simulink model "PSO_BON"  (R2019b)
settings: Solver=VariableStepAuto  StartTime=0.0  StopTime=0.2  RelTol=1e-5
undefined symbols (not defined in the file): sigbuilder_block
libraries: powerlib x164, re_lib x96, powerlib_meascontrol x9
(part 5 of 6)

== matlab function PSO_BON/Phasor PSO1/MATLAB Function1 ==
  settings: updateMethod=DISCRETE  sampleTime=1e-4
  data: Vpv input; Duty output; Ipv input
function Duty = PPSO(Vpv,Ipv)
coder.extrinsic('rand')
coder.extrinsic('format long')

persistent v_2 vmax_2 delta_2 iter_2 count_Part_2 count_2 pos_2 fitness_2 fitnessPbest_2 Pbest_2 fitnessGbest_2 Gbest_2 count_conv_2 reinit_2 Duty_Init_2;
Npart = 5;              % Nombre de particules de l'éssain
maxiter = 10000000;     % Nombre d'itération
% D = 1;                  % nombre d'espace de recherche

% Espace de recherche
% ------------------------------------
duty_cl_min = 0.1;      % Valeur minimale du rapport cyclique
duty_cl_max = 0.9;      % Valeur maximale du rapport cyclique

% Tolérance de la puissance
% ------------------------------------
tolerance = 1;          % Tolerance de la puissance en sortie

% Initialisation des vitesses des particules
% -------------------------------------------
if(isempty(vmax_2))
    vmax_2 = 0.5*(duty_cl_max - duty_cl_min);
end

if(isempty(v_2))
    v_2 = zeros(Npart,1);
end

% Initialisation de delta
% -------------------------------------------
if(isempty(delta_2))
    delta_2 = unifrnd(0,2*pi);
end

% Initialisation des positions des particules
% -------------------------------------------  
r = zeros(Npart,1);
r = rand(Npart,1);
if(isempty(pos_2))                                                          % Si la position des particules est inexistant
    pos_2 = zeros(Npart,1);
    for i = 1:Npart-2
        Min = duty_cl_min + (i-1)*(duty_cl_max-duty_cl_min)/(Npart-2);
        Max = Min + (duty_cl_max-duty_cl_min)/(Npart-2);
        pos_2(i+1) = Min + r(i)*(Max-Min);
%         pos_2(i) = duty_cl_min + ((duty_cl_max-duty_cl_min)*(i-1))/(Npart-1);
    end
    pos_2(1) = duty_cl_min;
    pos_2(Npart) = duty_cl_max;
end

% Initialisation des parametres persitents
% -------------------------------------------------
if(isempty(iter_2))       % Si le numéro de l'iteration est inexistant fixe à 1
    iter_2 = 1;
end

if(isempty(fitness_2))    % Si la fonction cout des particules est inexistant
    fitness_2 = zeros(Npart,1);
end

if(isempty(fitnessPbest_2))   % Si les fonctions couts des meilleures positions des particules est inexistant
    fitnessPbest_2 = zeros(Npart,1);
end

if(isempty(Pbest_2))      % Si les meilleures positions des particules est inexistant
    Pbest_2 = zeros(Npart,1);
end

if(isempty(Gbest_2))      % Si la meilleure position de l'éssain est inexistant
    Gbest_2 = zeros(maxiter,1);
end

if(isempty(fitnessGbest_2))   % Si la fonction cout de la meilleure position de l'éssain est inexistant
    fitnessGbest_2 = zeros(maxiter,1);
end

if(isempty(count_Part_2)) % Si le compteur de particule est inexistant
    count_Part_2 = 1;
end

if(isempty(count_conv_2)) % Si le compteur de particule convergente est inexistant
    count_conv_2 = zeros(Npart,1);
end

if(isempty(reinit_2))   % Si le coefficeint de reinitialisation est inexistant
    reinit_2 = 0;
end

if(isempty(Duty_Init_2))
    Duty_Init_2 = 0;
end

if(isempty(count_2))      % Si le compteur du régime transitoire est inexistant
    count_2 = 1;
end


% Evaluation des particules initiales
% -------------------------------------------------

%% phase transitoire d'évaluation d'une particule
% -------------------------------------------------
if (count_2 >= 1 && count_2 <= 20)
    Duty = pos_2(count_Part_2);
    count_2 = count_2 + 1;

    %% En cas de convergence
    % ---------------------------------------------
    if (reinit_2 == 1)  
        fitnessGbest_2(iter_2) = Vpv*Ipv;
        Duty = Duty_Init_2;
            if (abs(fitnessGbest_2(iter_2) - fitnessGbest_2(iter_2-1)) < 1)
                count_2 = count_2 - 1;
                reinit_2 = 1;
            else
                reinit_2 = 0;
                r = zeros(Npart,1);
                r = rand(Npart,1);
                pos_2 = zeros(Npart,1);
                for i = 1:Npart-2
                    Min = duty_cl_min + (i-1)*(duty_cl_max-duty_cl_min)/(Npart-2);
                    Max = Min + (duty_cl_max-duty_cl_min)/(Npart-2);
                    pos_2(i+1) = Min + r(i)*(Max-Min);
                end
                pos_2(1) = duty_cl_min;
                pos_2(Npart) = duty_cl_max;
                iter_2 = 0;
                vmax_2 = 0.5*(duty_cl_max - duty_cl_min);
                v_2 = zeros(Npart,1);
                delta_2 = unifrnd(0,2*pi);
                fitness_2 = zeros(Npart,1);
                fitnessPbest_2 = zeros(Npart,1);
                Pbest_2 = zeros(Npart,1);
                Gbest_2 = zeros(maxiter,1);
                fitnessGbest_2 = zeros(maxiter,1);
                count_Part_2 = 1;
                count_conv_2 = zeros(Npart,1);
                Duty_Init_2 = 0;
                count_2 = 1;
                iter_2 = iter_2 + 1;
            end 
    end
    return;
    
%%
else
    if(count_Part_2 <= (Npart - 1))
        Duty = pos_2(count_Part_2 + 1);
    else
        Duty = pos_2(1);
    end
end
                        % Programme PSO principale ou se fait la
                        % mise à jour des Pbest, de Gbest, des vitesse et
                        % des positions des particules
                        % -------------------------------------------------
fitness_2(count_Part_2) = Vpv*Ipv;  % Fonction cout des particules
if (count_Part_2 <= (Npart - 1))
    count_Part_2 = count_Part_2 + 1;
    count_2 = 2;
else
    if (iter_2 == 1)
                        % Initialisation des Pbest
                        % -------------------------------------------------
%         for j = 1:D
            for i = 1:Npart
                Pbest_2(i) = pos_2(i);
                fitnessPbest_2(i) = fitness_2(i);
            end
%         end
                        % Détermination de la fonction cout maximale
                        % -------------------------------------------------
        maxFitnessPbest = 0;
        FitnessPbest = fitnessPbest_2(:);
        for j = 1:length(FitnessPbest)
            if FitnessPbest(j) > maxFitnessPbest
                maxFitnessPbest = FitnessPbest(j);
            end
        end
                        % Initialisation de Gbest
                        % -------------------------------------------------
        fitnessGbest_2(iter_2) = maxFitnessPbest;
%         for i = 1:D
            for k = 1:Npart
                if(fitnessGbest_2(iter_2) == fitnessPbest_2(k))
                    Gbest_2(iter_2) = Pbest_2(k);
                end
            end
%         end
    elseif (iter_2 >= 2 && iter_2 <= maxiter)
                        % Mise à jour des Pbest
                        % -------------------------------------------------
%         for j = 1:D
            for i = 1:Npart
                if (fitness_2(i) > fitnessPbest_2(i))
                    Pbest_2(i) = pos_2(i);
                    fitnessPbest_2(i) = fitness_2(i);
                end
            end
%         end
                        % Mise à jour de Gbest
                        % -------------------------------------------------
        maxFitnessPbest = 0;
        FitnessPbest = fitnessPbest_2(:);
        for j = 1:length(FitnessPbest)
            if FitnessPbest(j) > maxFitnessPbest
                maxFitnessPbest = fitnessPbest_2(j);
            end
        end
        fitnessGbest_2(iter_2) = maxFitnessPbest;
%         for i = 1:D
            for k=1:Npart
                if(fitnessGbest_2(iter_2) == fitnessPbest_2(k))
                    Gbest_2(iter_2) = Pbest_2(k);
                end
            end
%         end
    end
                       % Test de convergence
                        % -------------------------------------------------
%     for j = 1:D
        for i = 1:Npart
            if ((fitnessGbest_2(iter_2) - fitnessPbest_2(i)) < tolerance)
                count_conv_2(i) = 1;
            end
        end
%     end
    n = sum(count_conv_2);
    if (n == Npart)
        reinit_2 = 1;
        Duty_Init_2 = Gbest_2(iter_2);
    else
        count_conv_2 = zeros(Npart,1);
    end
                        % Mise à jour des positions et des vitesses des
                        % particules
                        % -------------------------------------------------
        aa=2*(sin(delta_2));
        bb=2*(cos(delta_2));
        ee=abs(cos(delta_2))^aa;
        tt=abs(sin(delta_2))^bb;
    for i = 1:Npart
        v_2(i) = (ee)*(Pbest_2(i) - pos_2(i)) + (tt)*(Gbest_2(iter_2) - pos_2(i));
        if (v_2(i) > vmax_2)
            v_2(i) = vmax_2;
        end
        if (v_2(i) < -vmax_2)
            v_2(i) = -vmax_2;
        end
%         v_2(i) = min(max(v_2(i),-vmax_2),vmax_2);
        pos_2(i) = pos_2(i) + v_2(i);
        if (pos_2(i) > duty_cl_max)
            pos_2(i) = duty_cl_max;
        end
        if (pos_2(i) < duty_cl_min)
            pos_2(i) = duty_cl_min;
        end
%         pos_2(i) = min(max(pos_2(i),duty_cl_min),duty_cl_max);
    end
        delta_2 = delta_2 + (abs(aa + bb)*(2*pi));
        vmax_2 = (abs(cos(delta_2))^2)*(duty_cl_max - duty_cl_min);
                        % Mise à jour des positions et des vitesses
                        % -------------------------------------------------

                        % Contraindre la position mise à jour dans
                        % l'intervale de recherche
                        % -------------------------------------------------
%     end
    pos_2
    Duty = pos_2(1);
    count_Part_2 = 1;
    count_2 = 2;
    iter_2 = iter_2 + 1;
    if iter_2 > maxiter
        iter_2 = maxiter;
    end
end
end

== matlab function PSO_BON/Variant PSO1/MATLAB Function1 ==
  settings: updateMethod=DISCRETE  sampleTime=1e-4
  data: Vpv input; D output; Ipv input
function D = PSO(Vpv,Ipv)
%#codegen
persistent u;
persistent dcurrent;
persistent pbest;
persistent p;
persistent dc;
persistent v;
persistent counter;
persistent gbest;
Npart = 10;
if(isempty(counter))
    counter=0;
end
if(isempty(dcurrent))
    dcurrent=0.5;
end
if(isempty(gbest))
    gbest=0.5;
end
if(isempty(p))
    p=zeros(Npart,1);
end

if(isempty(v))
    v=zeros(Npart,1);
end

if(isempty(pbest))
    pbest=zeros(Npart,1);
end
if(isempty(u))
    u=0;
end
if(isempty(dc))
    dc=zeros(Npart,1);
    dc(1)=0;
    dc(2)=0.1;
    dc(3)=0.2;
    dc(4)=0.3;
    dc(5)=0.4;
    dc(6)=0.5;
    dc(7)=0.6;
    dc(8)=0.7;
    dc(9)=0.8;
    dc(10)=0.9;
end
if(counter>=1 && counter<20)
    D=dcurrent;
    counter=counter+1;
    return;
end
counter=0;

if(u>=1 && u<=Npart)
    if((Vpv*Ipv)>p(u))
        p(u)=Vpv*Ipv;
        pbest(u)=dcurrent;
    end
end
u=u+1;
if(u==Npart+2)
    u=1;
end
if(u==1)
    D=dc(u);
    dcurrent=D;
    counter=1;
    return;
elseif(u==2)
    D=dc(u);
    dcurrent=D;
    counter=1;
    return;
elseif(u==3)
    D=dc(u);
    dcurrent=D;
    counter=1;
    return;
elseif(u==4)
    D=dc(u);
    dcurrent=D;
    counter=1;
    return;
elseif(u==5)
    D=dc(u);
    dcurrent=D;
    counter=1;
    return;
elseif(u==6)
    D=dc(u);
    dcurrent=D;
    counter=1;
    return;
elseif(u==7)
    D=dc(u);
    dcurrent=D;
    counter=1;
    return;
elseif(u==8)
    D=dc(u);
    dcurrent=D;
    counter=1;
    return;
elseif(u==9)
    D=dc(u);
    dcurrent=D;
    counter=1;
    return;
elseif(u==10)
    D=dc(u);
    dcurrent=D;
    counter=1;
    return;
elseif(u==Npart+1)
    [m,i]=max(p);
    gbest=pbest(i);
    D=gbest;
    dcurrent=D;
    counter=1;
    %update velocity and duty cycle
    v(1)=updatevelocity(v(1),pbest(1),dc(1),gbest)
    v(2)=updatevelocity(v(2),pbest(2),dc(2),gbest)
    v(3)=updatevelocity(v(3),pbest(3),dc(3),gbest)
    v(4)=updatevelocity(v(4),pbest(4),dc(4),gbest)
    v(5)=updatevelocity(v(5),pbest(5),dc(5),gbest)
    v(6)=updatevelocity(v(6),pbest(6),dc(6),gbest)
    v(7)=updatevelocity(v(7),pbest(7),dc(7),gbest)
    v(8)=updatevelocity(v(8),pbest(8),dc(8),gbest)
    v(9)=updatevelocity(v(9),pbest(9),dc(9),gbest)
    v(10)=updatevelocity(v(10),pbest(10),dc(10),gbest)
    %update duty cycle
    dc(1)=updateduty(dc(1),v(1))
    dc(2)=updateduty(dc(2),v(2))
    dc(3)=updateduty(dc(3),v(3))
    dc(4)=updateduty(dc(4),v(4))
    dc(5)=updateduty(dc(5),v(5))
    dc(6)=updateduty(dc(6),v(6))
    dc(7)=updateduty(dc(7),v(7))
    dc(8)=updateduty(dc(8),v(8))
    dc(9)=updateduty(dc(9),v(9))
    dc(10)=updateduty(dc(10),v(10))
    return;
    
else
    u
    y='hello'
    D=0.1
    
end


end
function vfinal=updatevelocity(velocity,pobest,d,gwbest)
% PSO Parameters
w=0.4;
c1=1.2;       % Personal Learning Coefficient
c2=2;         % Global Learning Coefficient
beta = 1.5;
%w=(1.1-(pobest/gwbest));            % Inertia Weight
             % Inertia Weight Damping Ratio
% If you would like to use Constriction Coefficients for PSO,
% uncomment the following block and comment the above set of parameters.

% % Constriction Coefficients
% phi1=2.05;
% phi2=2.05;
% phi=phi1+phi2;
% chi=2/(phi-2+sqrt(phi^2-4*phi));
% w=chi;          % Inertia Weight
% wdamp=1;        % Inertia Weight Damping Ratio
% c1=chi*phi1;    % Personal Learning Coefficient
% c2=chi*phi2;    % Global Learning Coefficient
% vfinal = (w*velocity)+(c1*rand(1)*(pobest-d))+(c2*rand(1)*(gwbest-d));
vfinal = (w*velocity)+beta*(gwbest-d);
end
function dfinal=updateduty(d,velocity)
dup=d+velocity;
if(dup>0.9)
    dfinal=0.9;
elseif(dup<0.1)
    dfinal=0.1;
else
    dfinal=dup;
end
end

== matlab function PSO_BON/Phasor PSO1/MATLAB Function2 ==
  settings: updateMethod=DISCRETE  sampleTime=1e-4
  data: Vpv input; D output; Ipv input; G output; P output; Pow output; Powb output; Pp output
function [D, G, P, Pow, Powb, Pp] = PSO_Mod(Vpv,Ipv)
coder.extrinsic('rand')
coder.extrinsic('format long')

persistent iter count_Part count pos fitness fitnessPbest Pbest fitnessGbest Gbest count_conv reinit Duty_Init;
Npart = 5;              % Nombre de particules de l'éssain
maxiter = 10000000;           % Nombre d'itération

% Espace de recherche
% ------------------------------------
duty_cl_min = 0.1;      % Valeur minimale du rapport cyclique
duty_cl_max = 0.9;      % Valeur maximale du rapport cyclique

% Tolérance de la puissance
% ------------------------------------
tolerance = 1;          % Tolerance de la puissance en sortie

% Initialisation des positions des particules
% ------------------------------------
r = zeros(Npart,1);     % génération d'un vecteur de nombre aléatoire compris entre 0 et 1
r = rand(Npart,1);      
if(isempty(pos))        % Si la position des particules est inexistant
    pos = zeros(Npart,1);
%     for i = 1:Npart
%         pos(i) = duty_cl_min + ((duty_cl_max-duty_cl_min)*(i-1))/(Npart-1);
% %         pos(i) = duty_cl_min + r(i)*(duty_cl_max-duty_cl_min);
%     end
    
    for i = 1:Npart-2
        Min = duty_cl_min + (i-1)*(duty_cl_max-duty_cl_min)/(Npart-2);
        Max = Min + (duty_cl_max-duty_cl_min)/(Npart-2);
        pos(i+1) = Min + r(i)*(Max-Min);
    end
    pos(1) = duty_cl_min;
    pos(Npart) = duty_cl_max;
    Pp = pos;
end

% Initialisation des parametres persitents
% -------------------------------------------------
if(isempty(iter))       % Si le numéro de l'iteration est inexistant fixe à 1
    iter = 1;
end
if(isempty(fitness))    % Si la fonction cout des particules est inexistant
    fitness = zeros(Npart,1);
end
if(isempty(fitnessPbest))   % Si les fonctions couts des meilleures positions des particules est inexistant
    fitnessPbest = zeros(Npart,1);
    Powb = fitnessPbest;
end
if(isempty(Pbest))      % Si les meilleures positions des particules est inexistant
    Pbest = zeros(Npart,1);
    P = Pbest;
end
if(isempty(Gbest))      % Si la meilleure position de l'éssain est inexistant
    Gbest = zeros(maxiter,1);
end
if(isempty(fitnessGbest))   % Si la fonction cout de la meilleure position de l'éssain est inexistant
    fitnessGbest = zeros(maxiter,1);
    Pow = fitnessGbest(iter);
end
if(isempty(count_Part)) % Si le compteur de particule est inexistant
    count_Part = 1;
end
if(isempty(count_conv)) % Si le compteur de particule convergente est inexistant
    count_conv = zeros(Npart,1);
end
if(isempty(reinit))   % Si le coefficeint de reinitialisation est inexistant
    reinit = 0;
end
if(isempty(Duty_Init))
    Duty_Init = 0;
end
if(isempty(count))      % Si le compteur du régime transitoire est inexistant
    count = 1;
end

% Evaluation des particules initiales
% -------------------------------------------------

%% phase transitoire d'évaluation d'une particule
% -------------------------------------------------
if (count >= 1 && count <= 20)
    D = pos(count_Part);
    G = Duty_Init;
    P = Pbest;
    Pow = fitnessGbest(iter);
    Powb = fitnessPbest;
    Pp = pos;
    count = count + 1;

    %% En cas de convergence
    % ---------------------------------------------
    if (reinit == 1)  
        fitnessGbest(iter) = Vpv*Ipv;
        D = Duty_Init;
        G = Duty_Init;
        P = Pbest;
        Pp = pos;
        iter;
        Pow = fitnessGbest(iter);
        Powb = fitnessPbest;
%         if iter < 15
            if (abs(fitnessGbest(iter) - fitnessGbest(iter-1)) < 1)
                count = count - 1;
                iter;
                reinit = 1;
                Pow = fitnessGbest(iter);
                Powb = fitnessPbest;
                Pp = pos;
                P = Pbest;
            else
                reinit = 0;
                pos = zeros(Npart,1);    
                for i = 1:Npart-2
                    Min = duty_cl_min + (i-1)*(duty_cl_max-duty_cl_min)/(Npart-2);
                    Max = Min + (duty_cl_max-duty_cl_min)/(Npart-2);
                pos(i+1) = Min + r(i)*(Max-Min);
                end
                pos(1) = duty_cl_min;
                pos(Npart) = duty_cl_max;
                Pp = pos;
                P = Pbest;
                iter = 1;
                fitness = zeros(Npart,1);
                fitnessPbest = zeros(Npart,1);
                Pbest = zeros(Npart,1);
                Gbest = zeros(maxiter,1);
                fitnessGbest = zeros(maxiter,1);
                count_Part = 1;
                count_conv = zeros(Npart,1);
                Duty_Init = 0;
                count = 1;
            end
%         else
%             if (abs(fitnessGbest(iter) - fitnessGbest(iter-10)) < 0.5)
%                 count = count - 1;
%                 reinit = 1;
%             else
%                 reinit = 0;
%                 pos = zeros(Npart,1);    
%                 for i = 1:Npart-2
%                     Min = duty_cl_min + (i-1)*(duty_cl_max-duty_cl_min)/(Npart-2);
%                     Max = Min + (duty_cl_max-duty_cl_min)/(Npart-2);
%                 pos(i+1) = Min + r(i)*(Max-Min);
%                 end
%                 pos(1) = duty_cl_min;
%                 pos(Npart) = duty_cl_max;
%                 Pp = pos;
%                 iter = 1;
%                 fitness = zeros(Npart,1);
%                 fitnessPbest = zeros(Npart,1);
%                 Pbest = zeros(Npart,1);
%                 Gbest = zeros(maxiter,1);
%                 fitnessGbest = zeros(maxiter,1);
%                 count_Part = 1;
%                 count_conv = zeros(Npart,1);
%                 Duty_Init = 0;
%                 count = 1;
%             end
%         end
%         iter = iter + 1;
%         G = 0;
%         GG = 1;
%         P = zeros(Npart,1);
%         Pp = pos;
%         count = count - 1;          % Décrémenter
        
    end
    return;
    
%%
else
    if(count_Part <= (Npart - 1))
        D = pos(count_Part + 1);
        G = Gbest(iter);
        P = Pbest;
        Pp = pos;
        Pow = fitnessGbest(iter);
        Powb = fitnessPbest;
    else
        D = pos(1);
        G = Gbest(iter);
        P = Pbest;
        Pp = pos;
        Pow = fitnessGbest(iter);
        Powb = fitnessPbest;
    end
end


Pp = pos;
                        % Programme PSO principale ou se fait la
                        % mise à jour des Pbest, de Gbest, des vitesse et
                        % des positions des particules
                        % -------------------------------------------------
fitness(count_Part) = Vpv*Ipv;  % Fonction cout des particules
if (count_Part <= (Npart - 1))
    count_Part = count_Part + 1;
    count = 2;
else
    pos;
    Pp = pos;
    if (iter == 1)
                        % Initialisation des Pbest
                        % -------------------------------------------------
        for i = 1:Npart
            Pbest(i) = pos(i);
            fitnessPbest(i) = fitness(i);
        end
        Pbest;
        fitnessPbest;
        P = Pbest;
        Pow = fitnessGbest(iter);
        Powb = fitnessPbest;
        Pp = pos;
                        % Détermination de la fonction cout maximale
                        % -------------------------------------------------
        maxFitnessPbest = 0;
        for j = 1:length(fitnessPbest)
            if fitnessPbest(j) > maxFitnessPbest
                maxFitnessPbest = fitnessPbest(j);
            end
        end
                        % Initialisation de Gbest
                        % -------------------------------------------------
        fitnessGbest(iter) = maxFitnessPbest;
        for k = 1:Npart
            if(fitnessGbest(iter) == fitnessPbest(k))
                Gbest(iter) = Pbest(k);
            end
        end
    elseif (iter >= 2 && iter <= maxiter)
                        % Mise à jour des Pbest
                        % -------------------------------------------------
        for i = 1:Npart
            if (fitness(i) > fitnessPbest(i))
                Pbest(i) = pos(i);
                fitnessPbest(i) = fitness(i);
            end
        end
        Pbest;
        fitnessPbest;
        P = Pbest;
        Pow = fitnessGbest(iter);
        Powb = fitnessPbest;
        Pp = pos;
                        % Mise à jour de Gbest
                        % -------------------------------------------------
        maxFitnessPbest = 0;
        for j = 1:length(fitnessPbest)
            if fitnessPbest(j) > maxFitnessPbest
                maxFitnessPbest = fitnessPbest(j);
            end
        end
        fitnessGbest(iter) = maxFitnessPbest;
        for k=1:Npart
            if(fitnessGbest(iter) == fitnessPbest(k))
                Gbest(iter) = Pbest(k);
%                 G = Gbest(iter);
            end
        end
    end
    G = Gbest(iter);
                       % Test de convergence
                        % -------------------------------------------------
    for i = 1:Npart
        if ((fitnessGbest(iter) - fitnessPbest(i)) < tolerance)
            count_conv(i) = 1;
        end
    end
    n = sum(count_conv);
    if (n == Npart)
        reinit = 1;
        Duty_Init = Gbest(iter);
        G = Gbest(iter);
    else
        count_conv = zeros(Npart,1);
        G = Gbest(iter);
    end
                        % Mise à jour des positions et des vitesses des
                        % particules
                        % -------------------------------------------------
    for i = 1:Npart
                        % Mise à jour des positions sur le principe de la
                        % dichotomie
                        % -------------------------------------------------
%         if Gbest(iter) == Pbest(i)
%             pos(i) = Pbest(i) + 0.001;
%         else
            pos(i) = (Gbest(iter)+pos(i))/2;
%         end
                        % Contraindre la position mise à jour dans
                        % l'intervale de recherche
                        % -------------------------------------------------
        if (pos(i) > duty_cl_max)
            pos(i) = duty_cl_max;
        end
        if (pos(i) < duty_cl_min)
            pos(i) = duty_cl_min;
        end
    end
    pos;
    D = pos(1);
    iter
    reinit
    G = Gbest(iter);
    P = Pbest
    Pow = fitnessGbest(iter)
    Powb = fitnessPbest
    Pp = pos;
    count_Part = 1;
    count = 2;
    iter = iter + 1;
    if iter > maxiter
        iter = maxiter;
    end
end
end

== matlab function PSO_BON/InCond1/MATLAB Function1 ==
  settings: updateMethod=DISCRETE  sampleTime=1e-4
  data: V input; D output; I input
% InCond
function D= InCond(V,I)
delta=0.005;
Dmax = 0.9;   %Maximum value for D
Dmin = 0.1;   %Minimum value for D

persistent V0 I0 D0;
if isempty(V0)
    V0=0; I0=0; D0=0.5;
end
%-------------------------------------
m=0;
dV=V-V0; dI=I-I0; 
if dV==0             % Si no hay cambio voltaje
	  if dI==0
		 m=D0;
	  else
		if dI>0
		  m=D0-delta;
		else
		  m=D0+delta;
		end
	  end
elseif	dI/dV==-(I/V)   %no hacer nada (MPP)
else                    %dI/dV~=-(I/V)
        if dI/dV>-(I/V) %dI/dV>-(I/V) (izquierda MPP)
           m=D0-delta;  %disminuir D
        else            %dI/dV<-(I/V) (derecha MPP)
           m=D0+delta;  %aumentar D
        end 
end
D=m;
%-------------------------------------
if D >= Dmax || D<= Dmin
    D=D0;
end
%-------------------------------------
D0=D;
V0=V;
I0=I;

== matlab function PSO_BON/InCond1/MATLAB Function2 ==
  settings: updateMethod=DISCRETE  sampleTime=1e-4
  data: Vpv input; Duty output; Ipv input
function Duty = PSO_2(Vpv,Ipv)
coder.extrinsic('rand')
coder.extrinsic('format long')

persistent v_4 iter_4 count_Part_4 count_4 pos_4 fitness_4 fitnessPbest_4 Pbest_4 fitnessGbest_4 Gbest_4 count_conv_4 reinit_4 Duty_Init_4;
Npart_4 = 3;              % Nombre de particules de l'éssain
maxiter = 10000000;     % Nombre d'itération

% Espace de recherche
% ------------------------------------
duty_cl_min = 0.1;      % Valeur minimale du rapport cyclique
duty_cl_max = 0.9;      % Valeur maximale du rapport cyclique

% Tolérance de la puissance
% ------------------------------------
tolerance = 1;          % Tolerance de la puissance en sortie

% Initialisation des vitesses des particules
% -------------------------------------------
if(isempty(v_4))
    v_4 = zeros(Npart_4,1);
end

% hybrid initialisation
% ---------------------  
r = zeros(Npart_4,1);
r = rand(Npart_4,1);
if(isempty(pos_4))                                                          % Si la position des particules est inexistant
    pos_4 = zeros(Npart_4,1);
    for i = 1:Npart_4-2
        Min = duty_cl_min + (i-1)*(duty_cl_max-duty_cl_min)/(Npart_4-2);
        Max = Min + (duty_cl_max-duty_cl_min)/(Npart_4-2);
        pos_4(i+1) = Min + r(i)*(Max-Min);
    end
    pos_4(1) = duty_cl_min;
    pos_4(Npart_4) = duty_cl_max;
end
% pos
% Initialisation des parametres persitents
% -------------------------------------------------
if(isempty(iter_4))       % Si le numéro de l'iteration est inexistant fixe à 1
    iter_4 = 1;
end
if(isempty(fitness_4))    % Si la fonction cout des particules est inexistant
    fitness_4 = zeros(Npart_4,1);
end
if(isempty(fitnessPbest_4))   % Si les fonctions couts des meilleures positions des particules est inexistant
    fitnessPbest_4 = zeros(Npart_4,1);
end
if(isempty(Pbest_4))      % Si les meilleures positions des particules est inexistant
    Pbest_4 = zeros(Npart_4,1);
end
if(isempty(Gbest_4))      % Si la meilleure position de l'éssain est inexistant
    Gbest_4 = zeros(maxiter,1);
end
if(isempty(fitnessGbest_4))   % Si la fonction cout de la meilleure position de l'éssain est inexistant
    fitnessGbest_4 = zeros(maxiter,1);
end
if(isempty(count_Part_4)) % Si le compteur de particule est inexistant
    count_Part_4 = 1;
end
if(isempty(count_conv_4)) % Si le compteur de particule convergente est inexistant
    count_conv_4 = zeros(Npart_4,1);
end
if(isempty(reinit_4))   % Si le coefficeint de reinitialisation est inexistant
    reinit_4 = 0;
end
if(isempty(Duty_Init_4))
    Duty_Init_4 = 0;
end
if(isempty(count_4))      % Si le compteur du régime transitoire est inexistant
    count_4 = 1;
end


% Evaluation des particules initiales
% -------------------------------------------------

%% phase transitoire d'évaluation d'une particule
% -------------------------------------------------
if (count_4 >= 1 && count_4 <= 20)
    Duty = pos_4(count_Part_4);
    count_4 = count_4 + 1;

    %% En cas de convergence
    % ---------------------------------------------
    if (reinit_4 == 1)  
        fitnessGbest_4(iter_4) = Vpv*Ipv;
        Duty = Duty_Init_4;
       	if (abs(fitnessGbest_4(iter_4) - fitnessGbest_4(iter_4-1)) < 1)
         	count_4 = count_4 - 1;
           	reinit_4 = 1;
        else
          	reinit_4 = 0;
          	v_4 = zeros(Npart_4,1);
            r = zeros(Npart_4,1);
            r = rand(Npart_4,1);
           	pos_4 = zeros(Npart_4,1);
            for i = 1:Npart_4-2
                Min = duty_cl_min + (i-1)*(duty_cl_max-duty_cl_min)/(Npart_4-2);
                Max = Min + (duty_cl_max-duty_cl_min)/(Npart_4-2);
                pos_4(i+1) = Min + r(i)*(Max-Min);
            end
            pos_4(1) = duty_cl_min;
            pos_4(Npart_4) = duty_cl_max;
          	iter_4 = 0;
           	fitness_4 = zeros(Npart_4,1);
           	fitnessPbest_4 = zeros(Npart_4,1);
           	Pbest_4 = zeros(Npart_4,1);
           	Gbest_4 = zeros(maxiter,1);
            fitnessGbest_4 = zeros(maxiter,1);
           	count_Part_4 = 1;
           	count_conv_4 = zeros(Npart_4,1);
           	Duty_Init_4 = 0;
           	count_4 = 1;
          	iter_4 = iter_4 + 1;
        end
    end 
    return;
else
    if(count_Part_4 <= (Npart_4 - 1))
        Duty = pos_4(count_Part_4 + 1);
    else
        Duty = pos_4(1);
    end
end
                        % Programme PSO principale ou se fait la
                        % mise à jour des Pbest, de Gbest, des vitesse et
                        % des positions des particules
                        % -------------------------------------------------
fitness_4(count_Part_4) = Vpv*Ipv;  % Fonction cout des particules
if (count_Part_4 <= (Npart_4 - 1))
    count_Part_4 = count_Part_4 + 1;
    count_4 = 2;
else
%     nnn = 1;
    if (iter_4 == 1)
                        % Initialisation des Pbest
                        % -------------------------------------------------
            for i = 1:Npart_4
                Pbest_4(i) = pos_4(i);
                fitnessPbest_4(i) = fitness_4(i);
            end
                        % Détermination de la fonction cout maximale
                        % -------------------------------------------------
        maxFitnessPbest = 0;
        for j = 1:length(fitnessPbest_4)
            if fitnessPbest_4(j) > maxFitnessPbest
                maxFitnessPbest = fitnessPbest_4(j);
            end
        end
                        % Initialisation de Gbest
                        % -------------------------------------------------
        fitnessGbest_4(iter_4) = maxFitnessPbest;
            for k = 1:Npart_4
                if(fitnessGbest_4(iter_4) == fitnessPbest_4(k))
                    Gbest_4(iter_4) = Pbest_4(k);
                end
            end
    elseif (iter_4 >= 2 && iter_4 <= maxiter)
                        % Mise à jour des Pbest
                        % -------------------------------------------------
            for i = 1:Npart_4
                if (fitness_4(i) > fitnessPbest_4(i))
                    Pbest_4(i) = pos_4(i);
                    fitnessPbest_4(i) = fitness_4(i);
                end
            end
                        % Mise à jour de Gbest
                        % -------------------------------------------------
        maxFitnessPbest = 0;
        for j = 1:length(fitnessPbest_4)
            if fitnessPbest_4(j) > maxFitnessPbest
                maxFitnessPbest = fitnessPbest_4(j);
            end
        end
        fitnessGbest_4(iter_4) = maxFitnessPbest;
            for k=1:Npart_4
                if(fitnessGbest_4(iter_4) == fitnessPbest_4(k))
                    Gbest_4(iter_4) = Pbest_4(k);
                end
            end
    end
                        % Test de convergence
                        % -------------------------------------------------
         for i = 1:Npart_4
            if ((fitnessGbest_4(iter_4) - fitnessPbest_4(i)) < tolerance)
                count_conv_4(i) = 1;
            end
         end
    n = sum(count_conv_4);
    if (n == Npart_4)
        reinit_4 = 1;
        Duty_Init_4 = Gbest_4(iter_4);
    else
        count_conv_4 = zeros(Npart_4,1);
    end
                        % Mise à jour des positions et des vitesses des
                        % particules
                        % -------------------------------------------------
        for i = 1:Npart_4
            v_4(i) = updatevelocity(v_4(i),Pbest_4(i),pos_4(i),Gbest_4(iter_4));
            pos_4(i) = updateduty(pos_4(i),v_4(i));
            if (pos_4(i) > duty_cl_max)
                pos_4(i) = duty_cl_max;
            end
            if (pos_4(i) < duty_cl_min)
                pos_4(i) = duty_cl_min;
            end
        end
                        % Mise à jour des positions et des vitesses
                        % -------------------------------------------------

                        % Contraindre la position mise à jour dans
                        % l'intervale de recherche
                        % -------------------------------------------------
    pos_4
    Duty = pos_4(1);
    count_Part_4 = 1;
    count_4 = 2;
    iter_4 = iter_4 + 1;
    if iter_4 > maxiter
        iter_4 = maxiter;
    end
end
end

function vfinal=updatevelocity(velocity,pobest,d,gwbest)

% w1 = 0.1;
% w2 = 0.2;
% w = ((w1 - w2)*(Maxiter - Iter))/Maxiter + w2;

% c1f = 0.0015;       % Personal Learning Coefficient
% c1i = 1;         % Global Learning Coefficient
% c1 = ((c1f - c1i)*(Iter))/Maxiter + c1i;

% c2f = 1.4;       % Personal Learning Coefficient
% c2i = 0.3;         % Global Learning Coefficient
% c2 = ((c2f - c2i)*(Iter))/Maxiter + c2i;
c1 = 0.8;
c2 = 0.8;
c3 = 0.8;
w = 0.01;
a = zeros(3,1);
a = rand(3,1);
vfinal = (w*velocity) + (c1*a(1)*(pobest-d))+(c2*a(2)*(gwbest-d))+(c3*a(3)*(gwbest-d)*(pobest-d));
% vfinal = (w*velocity)+beta*(gwbest-d);
end
function dfinal=updateduty(d,velocity)
dup=d+velocity;
if(dup>0.9)
    dfinal=0.9;
elseif(dup<0.1)
    dfinal=0.1;
else
    dfinal=dup;
end
end

== matlab function PSO_BON/Phasor PSO1/MATLAB Function3 ==
  settings: updateMethod=DISCRETE  sampleTime=1e-4
  data: Vpv input; Duty output; Ipv input
function Duty = PPSO(Vpv,Ipv)
coder.extrinsic('rand')
coder.extrinsic('format long')

persistent v vmax delta iter count_Part count pos fitness fitnessPbest Pbest fitnessGbest Gbest count_conv reinit Duty_Init;
Npart = 10;              % Nombre de particules de l'éssain
maxiter = 10000000;     % Nombre d'itération
D = 1;                  % nombre d'espace de recherche

% Espace de recherche
% ------------------------------------
duty_cl_min = 0.1;      % Valeur minimale du rapport cyclique
duty_cl_max = 0.9;      % Valeur maximale du rapport cyclique

% Tolérance de la puissance
% ------------------------------------
tolerance = 1;          % Tolerance de la puissance en sortie

% Initialisation des vitesses des particules
% -------------------------------------------
if(isempty(vmax))
    vmax = zeros(D,1);
for i = 1:D
    vmax(i) = 0.5*(duty_cl_max - duty_cl_min);
end
end

if(isempty(v))
    v = zeros(D,Npart);
end

% Initialisation de delta
% -------------------------------------------
if(isempty(delta))
    delta = zeros(D,1);
    for i = 1:D
        delta(i) = unifrnd(0,2*pi);
    end
end

% Initialisation des positions des particules
% -------------------------------------------  
r = zeros(Npart,1);
r = rand(Npart,1);
if(isempty(pos))        % Si la position des particules est inexistant
    pos = zeros(D,Npart);
    for i = 1:D
        for j = 1:Npart
        pos(i,j) = duty_cl_min + ((duty_cl_max-duty_cl_min)*(j-1))/(Npart-1);
%         pos(i,:) = duty_cl_min + r*(duty_cl_max-duty_cl_min);
        end
    end
end

% Initialisation des parametres persitents
% -------------------------------------------------
if(isempty(iter))       % Si le numéro de l'iteration est inexistant fixe à 1
    iter = 1;
end
if(isempty(fitness))    % Si la fonction cout des particules est inexistant
    fitness = zeros(D,Npart);
end
if(isempty(fitnessPbest))   % Si les fonctions couts des meilleures positions des particules est inexistant
    fitnessPbest = zeros(D,Npart);
end
if(isempty(Pbest))      % Si les meilleures positions des particules est inexistant
    Pbest = zeros(D,Npart);
end
if(isempty(Gbest))      % Si la meilleure position de l'éssain est inexistant
    Gbest = zeros(maxiter,1);
end
if(isempty(fitnessGbest))   % Si la fonction cout de la meilleure position de l'éssain est inexistant
    fitnessGbest = zeros(maxiter,1);
end
if(isempty(count_Part)) % Si le compteur de particule est inexistant
    count_Part = 1;
end
if(isempty(count_conv)) % Si le compteur de particule convergente est inexistant
    count_conv = zeros(D,Npart);
end
if(isempty(reinit))   % Si le coefficeint de reinitialisation est inexistant
    reinit = 0;
end
if(isempty(Duty_Init))
    Duty_Init = 0;
end
if(isempty(count))      % Si le compteur du régime transitoire est inexistant
    count = 1;
end


% Evaluation des particules initiales
% -------------------------------------------------

%% phase transitoire d'évaluation d'une particule
% -------------------------------------------------
if (count >= 1 && count <= 20)
    Duty = pos(count_Part);
    count = count + 1;

    %% En cas de convergence
    % ---------------------------------------------
    if (reinit == 1)  
        fitnessGbest(iter) = Vpv*Ipv;
        Duty = Duty_Init;
            if (abs(fitnessGbest(iter) - fitnessGbest(iter-1)) < 1)
                count = count - 1;
                reinit = 1;
            else
                reinit = 0;
                r = zeros(Npart,1);
                r = rand(Npart,1);
%                 if(isempty(pos))        % Si la position des particules est inexistant
                    pos = zeros(D,Npart);
                    for i = 1:D
                        for j = 1:Npart
                        pos(i,j) = duty_cl_min + ((duty_cl_max-duty_cl_min)*(j-1))/(Npart-1);
                %         pos(i,:) = duty_cl_min + r*(duty_cl_max-duty_cl_min);
                        end
                    end
%                 end
                iter = 0;
%                 if(isempty(vmax))
                    vmax = zeros(D,1);
                for i = 1:D
                    vmax(i) = 0.5*(duty_cl_max - duty_cl_min);
                end
%                 end

%                 if(isempty(v))
                    v = zeros(D,Npart);
%                 end

                % Initialisation de delta
                % -------------------------------------------
%                 if(isempty(delta))
                    delta = zeros(D,1);
                    for i = 1:D
                        delta(i) = unifrnd(0,2*pi);
                    end
%                 end

                fitness = zeros(D,Npart);
                fitnessPbest = zeros(D,Npart);
                Pbest = zeros(D,Npart);
                Gbest = zeros(maxiter,1);
                fitnessGbest = zeros(maxiter,1);
                count_Part = 1;
                count_conv = zeros(D,Npart);
                Duty_Init = 0;
                count = 1;
                iter = iter + 1;
            end 
    end
    return;
    
%%
else
    if(count_Part <= (Npart - 1))
        Duty = pos(count_Part + 1);
    else
        Duty = pos(1);
    end
end
                        % Programme PSO principale ou se fait la
                        % mise à jour des Pbest, de Gbest, des vitesse et
                        % des positions des particules
                        % -------------------------------------------------
fitness(count_Part) = Vpv*Ipv;  % Fonction cout des particules
if (count_Part <= (Npart - 1))
    count_Part = count_Part + 1;
    count = 2;
else
    if (iter == 1)
                        % Initialisation des Pbest
                        % -------------------------------------------------
        for j = 1:D
            for i = 1:Npart
                Pbest(j,i) = pos(j,i);
                fitnessPbest(j,i) = fitness(j,i);
            end
        end
                        % Détermination de la fonction cout maximale
                        % -------------------------------------------------
        maxFitnessPbest = 0;
        FitnessPbest = fitnessPbest(:);
        for j = 1:length(FitnessPbest)
            if FitnessPbest(j) > maxFitnessPbest
                maxFitnessPbest = FitnessPbest(j);
            end
        end
                        % Initialisation de Gbest
                        % -------------------------------------------------
        fitnessGbest(iter) = maxFitnessPbest;
        for i = 1:D
            for k = 1:Npart
                if(fitnessGbest(iter) == fitnessPbest(i,k))
                    Gbest(iter) = Pbest(i,k);
                end
            end
        end
    elseif (iter >= 2 && iter <= maxiter)
                        % Mise à jour des Pbest
                        % -------------------------------------------------
        for j = 1:D
            for i = 1:Npart
                if (fitness(j,i) > fitnessPbest(j,i))
                    Pbest(j,i) = pos(j,i);
                    fitnessPbest(j,i) = fitness(j,i);
                end
            end
        end
                        % Mise à jour de Gbest
                        % -------------------------------------------------
        maxFitnessPbest = 0;
        FitnessPbest = fitnessPbest(:);
        for j = 1:length(FitnessPbest)
            if FitnessPbest(j) > maxFitnessPbest
                maxFitnessPbest = fitnessPbest(j);
            end
        end
        fitnessGbest(iter) = maxFitnessPbest;
        for i = 1:D
            for k=1:Npart
                if(fitnessGbest(iter) == fitnessPbest(i,k))
                    Gbest(iter) = Pbest(i,k);
                end
            end
        end
    end
                       % Test de convergence
                        % -------------------------------------------------
    for j = 1:D
        for i = 1:Npart
            if ((fitnessGbest(iter) - fitnessPbest(j,i)) < tolerance)
                count_conv(j,i) = 1;
            end
        end
    end
    n = sum(sum(count_conv));
    if (n == Npart*D)
        reinit = 1;
        Duty_Init = Gbest(iter);
    else
        count_conv = zeros(D,Npart);
    end
                        % Mise à jour des positions et des vitesses des
                        % particules
                        % -------------------------------------------------
    for i = 1:D
        aa=2*(sin(delta(i)));
        bb=2*(cos(delta(i)));
        ee=abs(cos(delta(i)))^aa;
        tt=abs(sin(delta(i)))^bb;
        
        v(i,:) = (ee)*(Pbest(i,:) - pos(i,:)) + (tt)*(Gbest(iter) - pos(i,:));
        v(i,:) = min(max(v(i,:),-vmax(i)),vmax(i));
        pos(i,:) = pos(i,:) + v(i,:);
        pos(i,:) = min(max(pos(i,:),duty_cl_min),duty_cl_max);
        delta(i) = delta(i)+(abs(aa + bb)*(2*pi));
        vmax(i) = (abs(cos(delta(i)))^2)*(duty_cl_max - duty_cl_min);
                        % Mise à jour des positions et des vitesses
                        % -------------------------------------------------

                        % Contraindre la position mise à jour dans
                        % l'intervale de recherche
                        % -------------------------------------------------
    end
    Duty = pos(1);
    count_Part = 1;
    count = 2;
    iter = iter + 1;
    if iter > maxiter
        iter = maxiter;
    end
end
end
